simulink model "LabB_ControllerOverSimulator_Discrete"  (R2017a)
settings: Solver=FixedStepAuto  StartTime=0.0  StopTime=5  FixedStep=0.001  RelTol=1e-3
values from neighbouring files (symbols this model uses):
  Kd = [-8.1792  -49.1223  -71.4928  -11.5909]    [LabB_ControllerOverSimulator_Discrete_Parameters.m]
undefined symbols (not defined in the file or in its folder): sigbuilder_block
Description:
  | Real-Time Van der Pol Simulation
  | 
  | This model shows a real-time version of the Simulink(R) Van der Pol
  | simulation model. This model does not need any external signals, so it does
  | not need any data acquisition hardware or driver. This makes the model ideal
  | for first experiments with Simulink Desktop Real-Time(TM), without need to
  | worry about proper I/O hardware configuration.
  | 
  | How to run this model in Normal Mode:
  | 
  | 1) Double-click the orange button to switch to Normal Mode if needed.
  | 2) Start the real-time execution using Simulation->Run.
  | 3) Observe any missed ticks on the Missed Ticks scope.
  | 
  | How to run this model in External Mode:
  | 
  | 1) Double-click the orange button to switch to External Mode if needed.
  | 2) Start the real-time execution using Simulation->Run. The model will automatically
  |    build, connect to Simulink in External Mode and start.
  | 3) Missed ticks will be always zero.
settings Model: ExtModeTrigDuration=101  Creator=The MathWorks Inc.  LastModifiedBy=damiano
settings DataIOCC: LimitDataPoints=on  SaveFormat=Array  SignalLoggingName=logsOut
settings OptimizationCC: ExpressionDepthLimit=2147483647  InitFltsAndDblsToZero=on  EfficientMapNaN2IntZero=off
settings DebuggingCC: UnderspecifiedInitializationDetection=Classic  MergeDetectMultiDrivingBlocksExec=none  SignalResolutionControl=TryResolveAllWithWarning  FcnCallInpInsideContextMsg=warning  StateNameClashWarn=warning  SFUnexpectedBacktrackingDiag=warning  SFNoUnconditionalDefaultTransitionDiag=warning  SFExecutionAtInitializationDiag=none
settings HardwareCC: TargetBitPerLong=64  TargetBitPerPointer=64  TargetIntDivRoundTo=Zero  TargetEndianess=LittleEndian  TargetWordSize=64  TargetHWDeviceType=Intel->x86-64
settings ModelReferenceCC: PropagateSignalLabelsOutOfModel=off
settings RTWCC: SystemTargetFile=sldrt.tlc  TemplateMakefile=sldrt.tmf  Description=Simulink Desktop Real-Time  RTWCompilerOptimization=on
settings CodeAppCC: MaxIdLength=95
settings SimulinkDesktopRealTimeCC: TargetPreCompLibLocation=C:\Program Files\MATLAB\R2017a\toolbox\sldrt\lib\win64  TargetLangStandard=C89/C90 (ANSI)  SupportVariableSizeSignals=off
settings ConfigComp: CovMetricSettings=dw  CovHtmlReporting=on  CovSaveCumulativeToWorkspaceVar=on  CovSaveSingleToWorkspaceVar=on  CovExternalEMLEnable=off  CovSFcnEnable=off

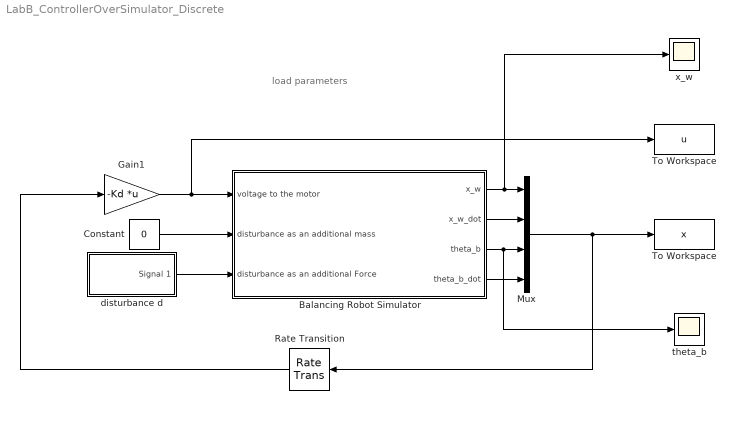
== system LabB_ControllerOverSimulator_Discrete ==
  note: load parameters
  Balancing Robot Simulator : Subsystem  mask(Balancing Robot Simulator Parameters){g=9.8, m_b=0.381, l_b=0.112, I_b=0.00616, m_w=0.036, l_w=0.021, I_w=0.00000746, R_m=4.4, L_m=0, b_m=0, b_f=0, K_e=0.444, K_t=0.470, X_0=0, x_w=0.011357, Theta=0.0001473, circle_x=0, circle_y=0, scale=2, v_m_limit=9, Theta_0=0*pi/180, x_w_0=0, sigma2_angle=0}
      mask prompts: g "gravitational acceleration"; m_b "mass of the body [kg]"; l_b "length of the body [m]"; I_b "moment of inertia of the body [kg m^2]"; m_w "mass of the wheels [kg]"; l_w "radius of the wheels [m]"; I_w "moment of inertia of the wheels [kg m^2]"; R_m "electrical resistance of the motor [Ohm]"; L_m "electrical inductance of the motor [Henry]"; b_m "viscuous coefficient of the motor"; b_f "wheels - ground friction coefficient"; K_e "back EMF constant of the motor"; K_t "torque constant of the motor"; circle_x "Circl_x"; circle_y "Circl_y"; v_m_limit "saturation limits for the motor voltage"; Theta_0 "initial angle of the body"; x_w_0 "initial position of the wheels"; sigma2_angle "variance of the angle measurement noise"
      mask init:
      | hBlk=get_param(gcb,'Handle');
      | 
      | X_0=[Theta_0 0 x_w_0 0];
      | %%% calculate the circle
      | 
      | r=l_w ;
      | x=-r:r/10:r;
      | circle_y=r*[sqrt(1-x.^2/r^2), -sqrt(1-x.^2/r^2) ]+r;
      | circle_x=[x,x([length(x):-1:1])];
      mask Display:
      | color('black');
      | plot([0.0,0.0,1 ,1,0 ],[1,0,0,1,1])
      | port_label('input',		1,  'motor voltage')
      | port_label('input',		2,  'additional mass')
      | port_label('input',		3,  'additional force')
      | port_label('output',	1,	'x_w')
      | port_label('output',	2,	'x_w_dot')
      | port_label('output',	3,	'theta_b')
      | port_label('output',	4,	'theta_b_dot')
      | 
      | x_b = x_w + l_b * sin(Theta);
      | y_b = l_w + l_b * cos(Theta);
      | 
      | Y_OFF = 0.1;
      | X_OFF = 0.5;
      | 
      | plot([0.05,0.95],[Y_OFF,Y_OFF])
      | plot([0.5,0.5],[Y_OFF/2,Y_OFF])
      | 
      | color('r');
      | plot(	(circle_x+x_w)*scale +X_OFF,	...
      | 		(circle_y)*scale+Y_OFF			);
      | 
      | plot(	[x_w x_b] * scale + X_OFF,	...
      | 		[l_w y_b] * scale + Y_OFF	);
      | 
      | color('r');
      | text(0.5, 0.5,																	...
      | 	['theta_b = ' num2str(Theta*180/pi,3) char(10) 'x_w = ' num2str(x_w,3)],		...
      | 	'HorizontalAlignment',	'center',											...
      |     'VerticalAlignment',	'bottom'											);
  Constant : Constant  Value=0
  Gain1 : Gain  Gain=-Kd  Multiplication=Matrix(K*u)
  Mux : Mux
  Rate Transition : RateTransition  OutPortSampleTime=fSamplingPeriod
  To Workspace : ToWorkspace  VariableName=x  SaveFormat=Structure With Time  SampleTime=-1
  "To Workspace " : ToWorkspace  VariableName=u  SaveFormat=Structure With Time  SampleTime=-1
  disturbance d : Subsystem  Tag=STV Subsys  LoadFcn=sigbuilder_block('load');  StartFcn=sigbuilder_block('start');  StopFcn=sigbuilder_block('stop');  ClipboardFcn=sigbuilder_block('clipboard');  mask(Sigbuilder block){tuvar=[0:10]}
      mask help: Simulink:masks:SigbuilderBlock_MD
      mask init:
      | if ~strcmp(get_param(bdroot(gcbh),'SimulationStatus'),'stopped') tuvar = sigbuilder_block('maskInit'); end
      settings: CopyFcn=sigbuilder_block('copy');  DeleteFcn=sigbuilder_block('delete');  ModelCloseFcn=sigbuilder_block('modelClose');  PreSaveFcn=sigbuilder_block('preSave');  PauseFcn=sigbuilder_block('pause');  ContinueFcn=sigbuilder_block('continue');  NameChangeFcn=sigbuilder_block('namechange');  OpenFcn=sigbuilder_block('open',[437.6 199.2 550.4 400 ]);  CloseFcn=sigbuilder_block('close');
      mask Display: plot(0, 0, 100, 100,[2, 2, 32, 32, 2], [68, 8, 8, 68, 68],[32, 2], [38, 38], [32, 19, 2],[53, 60, 44], [32, 17, 17, 2],[16, 16, 31, 31]);txt = getActiveGroup(gcbh);text(2, 100, txt,'verticalAlignment', 'top');
  theta_b : Scope
  x_w : Scope
  wires:
  disturbance d/1(Signal 1) -> Balancing Robot Simulator/3(disturbance as an additional Force)
  Balancing Robot Simulator/4("theta_b_dot ") -> Mux/4
  Balancing Robot Simulator/2(x_w_dot) -> Mux/2
  Rate Transition/1 -> Gain1/1
  Gain1/1 -> Balancing Robot Simulator/1(voltage to the motor), "To Workspace "/1
  Mux/1 -> To Workspace/1, Rate Transition/1
  Balancing Robot Simulator/3(theta_b) -> theta_b/1, Mux/3
  Balancing Robot Simulator/1(x_w) -> x_w/1, Mux/1
  Constant/1 -> Balancing Robot Simulator/2("disturbance as an additional mass ")

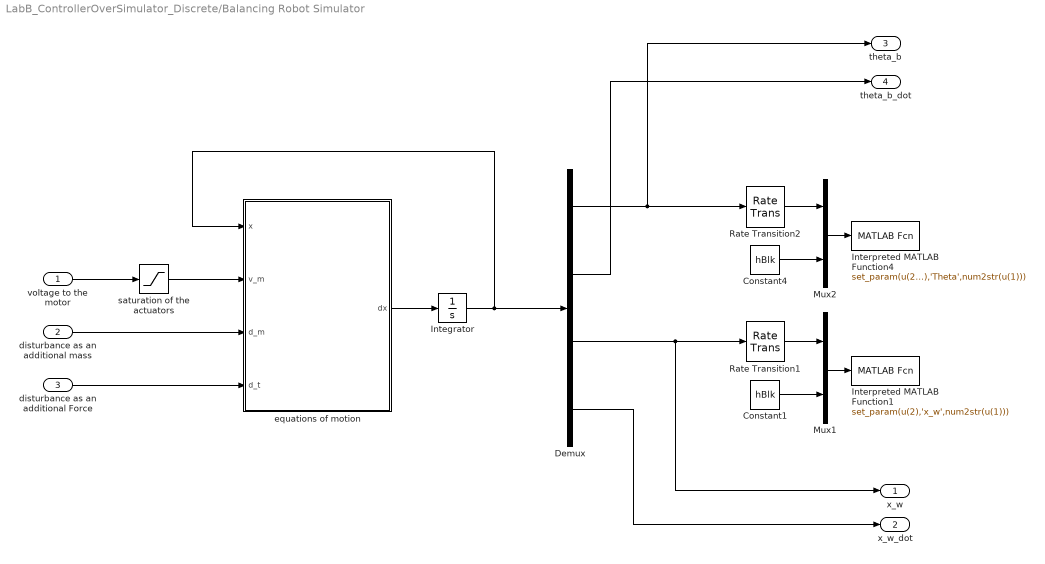
== system LabB_ControllerOverSimulator_Discrete/Balancing Robot Simulator ==
  voltage to the motor : Inport
  "disturbance as an additional mass " : Inport  Port=2
  disturbance as an additional Force : Inport  Port=3
  Constant1 : Constant  Value=hBlk
  Constant4 : Constant  Value=hBlk
  Demux : Demux
  Integrator : Integrator  InitialCondition=X_0
  Interpreted MATLAB Function1 : MATLABFcn  MATLABFcn=set_param(u(2),'x_w',num2str(u(1)))  OutputDimensions=0  SampleTime=0.1
  Interpreted MATLAB Function4 : MATLABFcn  MATLABFcn=set_param(u(2),'Theta',num2str(u(1)))  OutputDimensions=0
  Mux1 : Mux  Inputs=2
  Mux2 : Mux  Inputs=2
  Rate Transition1 : RateTransition  OutPortSampleTime=0.1
  Rate Transition2 : RateTransition  OutPortSampleTime=0.1
  equations of motion : MATLAB Function  TreatAsAtomicUnit=on
  saturation of the actuators : Saturate  UpperLimit=v_m_limit  LowerLimit=-v_m_limit
  x_w : Outport
  x_w_dot : Outport  Port=2
  theta_b : Outport  Port=3
  "theta_b_dot " : Outport  Port=4
  wires:
  Integrator/1 -> equations of motion/1(x), Demux/1
  Constant4/1 -> Mux2/2
  Mux2/1 -> Interpreted MATLAB Function4/1
  Rate Transition2/1 -> Mux2/1
  equations of motion/1(dx) -> Integrator/1
  voltage to the motor/1 -> saturation of the actuators/1
  Constant1/1 -> Mux1/2
  Mux1/1 -> Interpreted MATLAB Function1/1
  Rate Transition1/1 -> Mux1/1
  Demux/3 -> x_w/1, Rate Transition1/1
  saturation of the actuators/1 -> equations of motion/2(v_m)
  "disturbance as an additional mass "/1 -> equations of motion/3(d_m)
  disturbance as an additional Force/1 -> equations of motion/4(d_t)
  Demux/1 -> theta_b/1, Rate Transition2/1
  Demux/2 -> "theta_b_dot "/1
  Demux/4 -> x_w_dot/1

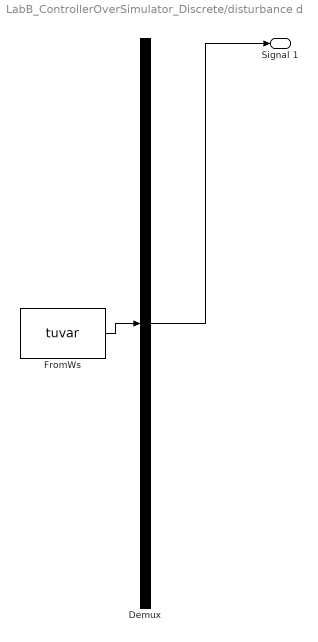
== system LabB_ControllerOverSimulator_Discrete/disturbance d ==
  Demux : Demux  Tag=STV Demux  Outputs=1
  FromWs : FromWorkspace  Tag=STV FromWs  VariableName=tuvar  SampleTime=0
      SigBuilderData=|
      | common.afterFinalStr = 'Extrapolate'
      | common.sampleTime = 0
      | dataSet.timeRange = [0 10]
      | dataSet.name = 'Group 1'
      | sbobj.Groups.Name = 'Group 1'
      | sbobj.Groups.Signals.Name = 'Signal 1'
      | sbobj.Groups.Signals.XData = [0 0.1 0.1 10]
      | sbobj.Groups.Signals.YData = [0.6 0.6 0 0]
  Signal 1 : Outport  Tag=STV Outport
  wires:
  Demux/1 -> Signal 1/1
  FromWs/1 -> Demux/1

== matlab function LabB_ControllerOverSimulator_Discrete/Balancing Robot Simulator/equations of motion ==
  data: x input; dx output; v_m input; d_m input; d_t input; g parameter; b_f parameter; m_b parameter; l_b parameter; I_b parameter; m_w parameter; l_w parameter; I_w parameter; R_m parameter; L_m parameter; b_m parameter; K_e parameter; K_t parameter
function dx = EquationsOfMotion(x,		...
								v_m,	...
								d_m,	... % additional mass on the body
								d_t,	... % Fource that acted on the body
								g,		...
								b_f,	...
								m_b,	...
								l_b,	...
								I_b,	...
								m_w,	...
								l_w,	...
								I_w,	...
								R_m,	...
								L_m,	...
								b_m,	...
								K_e,	...
								K_t		) %#ok<*INUSL>

% initialization of the state
dx = zeros(4,1);

% TODO: the motor electrical inductance and the motor viscous coefficients
% are neglected

% for readability -- state of the system
theta		= x(1);
theta_dot	= x(2);
x_b			= x(3);
x_b_dot		= x(4);

% add the mass disturbance: notice that we need to modify also the
% moment of inertia
m_t_b = m_b + d_m;
I_t_b = I_b * m_t_b / m_b;

% equations of motion (obfuscated)
dx(1)=theta_dot;
dx(2)=((b_f + (K_e*K_t)/R_m)*(theta_dot - x_b_dot/l_w) + (K_t*v_m)/R_m - d_t*l_b*1*cos(theta) - g*l_b*m_t_b*sin(theta) + (l_b*m_t_b*cos(theta)*(d_t*l_w + (b_f + (K_e*K_t)/R_m)*(theta_dot - x_b_dot/l_w) + (K_t*v_m)/R_m + l_b*l_w*m_t_b*theta_dot^2*sin(theta)))/(l_w*m_t_b + l_w*m_w + I_w/l_w))/((m_t_b*l_b^2 + I_t_b)*((l_b^2*l_w*m_t_b^2*cos(theta)^2)/((m_t_b*l_b^2 + I_t_b)*(l_w*m_t_b + l_w*m_w + I_w/l_w)) - 1));
dx(3)=x_b_dot;
dx(4)= -(d_t*l_w + (b_f + (K_e*K_t)/R_m)*(theta_dot - x_b_dot/l_w) + (K_t*v_m)/R_m + l_b*l_w*m_t_b*theta_dot^2*sin(theta) + (l_b*l_w*m_t_b*cos(theta)*((b_f + (K_e*K_t)/R_m)*(theta_dot - x_b_dot/l_w) + (K_t*v_m)/R_m - d_t*l_b*1*cos(theta) - g*l_b*m_t_b*sin(theta)))/(m_t_b*l_b^2 + I_t_b))/(((l_b^2*l_w*m_t_b^2*cos(theta)^2)/((m_t_b*l_b^2 + I_t_b)*(l_w*m_t_b + l_w*m_w + I_w/l_w)) - 1)*(l_w*m_t_b + l_w*m_w + I_w/l_w));

% if the robot falls
if( (x(1) > pi/2) || (x(1) < -pi/2) )
	%
	dx(1) = 0;
	dx(2) = 0;
	dx(3) = 0;
	dx(4) = 0;
	%
end;%


% g   = 9.8;
% b_f = 0;
% m_t_b = 0.381;
% l_b = 0.112;
% I_t_b = 0.00616;
% m_w = 0.036;
% l_w = 0.021;
% I_w = 0.00000746;
% R_m = 4.4;
% L_m = 0 ;
% b_m = 0;
% K_e = 0.444;
% K_t = 0.470;
